simulink model "functional_architecture"  (R2024b)
settings: Solver=VariableStepAuto  StartTime=0.0  StopTime=10.0  RelTol=1e-3
settings Model: Creator=upattacini  LastModifiedBy=mfussi
settings DataIOCC: SaveOutput=off  SignalLogging=off  DSMLogging=off  SaveTime=off
settings RTWCC: GPUComputeCapability=3.5

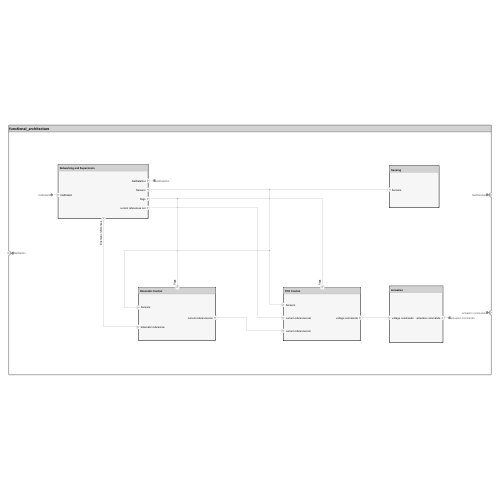
[thumbnail: Simulink's stored preview of the top-level diagram]
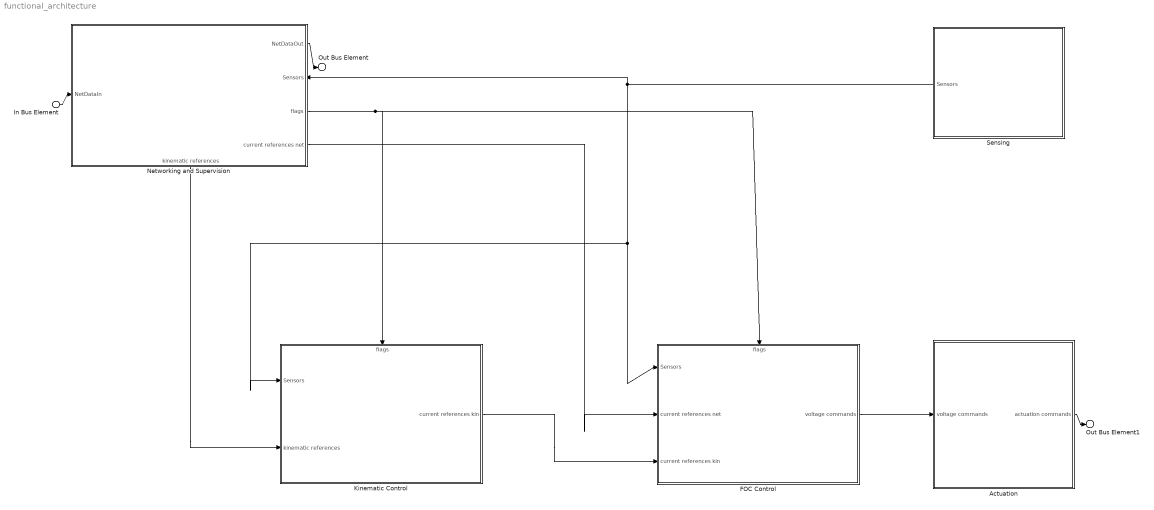
== system functional_architecture ==
  In Bus Element : Inport  PortName=NetDataIn
  Actuation : Subsystem
      settings: PortSchema="{\"entries\":[{\"content\":{\"headerSize\":26,\"margin\":15,\"minimumSpacing\":25,\"sides\":[{\"content\":{\"connectorIds\":[\"In1\"]},\"type\":\"ConnectorPlacement.EquallySpacedRectSide\",\"uuid\":\"e347ee40-d54e-44fd-bc32-f8b024d9ce0e\"},{\"content\":{\"connectorIds\":[\"Out1\"],\"side\":\"RIGHT\"},\"type\":\"ConnectorPlacement.EquallySpacedRectSide\",\"uuid\":\"0804b9f8-7204-402a-a199-b5abf958a170\"},{\"content\":{\"side\":\"TOP\"},\"type\":\"ConnectorPlacement.EquallySpacedRectSide\",\"uuid\":\"09180045-bcf9-4b06-aaa4-a03943964dca\"}]},\"type\":\"ConnectorPlacement.EquallySpacedConnector\",\"uuid\":\"bea07901-0638-4912-923c-a7a96e6d9f8d\"}],\"packageUris\":[\"http://schema.mathworks.com/mf0/Connector/R2020b\"],\"version\":\"1.0\"}"
  FOC Control : Subsystem
      settings: PortSchema="{\"entries\":[{\"content\":{\"headerSize\":26,\"margin\":15,\"minimumSpacing\":25,\"sides\":[{\"content\":{\"connectorIds\":[\"In3\",\"In2\",\"In4\"]},\"type\":\"ConnectorPlacement.EquallySpacedRectSide\",\"uuid\":\"e347ee40-d54e-44fd-bc32-f8b024d9ce0e\"},{\"content\":{\"connectorIds\":[\"Out1\"],\"side\":\"RIGHT\"},\"type\":\"ConnectorPlacement.EquallySpacedRectSide\",\"uuid\":\"0804b9f8-7204-402a-a199-b5abf958a170\"},{\"content\":{\"connectorIds\":[\"In1\"],\"side\":\"TOP\"},\"type\":\"ConnectorPlacement.EquallySpacedRectSide\",\"uuid\":\"09180045-bcf9-4b06-aaa4-a03943964dca\"},{\"content\":{\"side\":\"BOTTOM\"},\"type\":\"ConnectorPlacement.EquallySpacedRectSide\",\"uuid\":\"ba1d2f98-a278-4884-ad0d-7d0295f27101\"}]},\"type\":\"ConnectorPlacement.EquallySpacedConnector\",\"uuid\":\"bea07901-0638-4912-923c-a7a96e6d9f8d\"}],\"packageUris\":[\"http://schema.mathworks.com/mf0/Connector/R2020b\"],\"version\":\"1.0\"}"
  Kinematic Control : Subsystem
      settings: PortSchema="{\"entries\":[{\"content\":{\"headerSize\":26,\"margin\":15,\"minimumSpacing\":25,\"sides\":[{\"content\":{\"connectorIds\":[\"In2\",\"In3\"]},\"type\":\"ConnectorPlacement.EquallySpacedRectSide\",\"uuid\":\"e347ee40-d54e-44fd-bc32-f8b024d9ce0e\"},{\"content\":{\"connectorIds\":[\"Out1\"],\"side\":\"RIGHT\"},\"type\":\"ConnectorPlacement.EquallySpacedRectSide\",\"uuid\":\"0804b9f8-7204-402a-a199-b5abf958a170\"},{\"content\":{\"connectorIds\":[\"In1\"],\"side\":\"TOP\"},\"type\":\"ConnectorPlacement.EquallySpacedRectSide\",\"uuid\":\"09180045-bcf9-4b06-aaa4-a03943964dca\"},{\"content\":{\"side\":\"BOTTOM\"},\"type\":\"ConnectorPlacement.EquallySpacedRectSide\",\"uuid\":\"ba1d2f98-a278-4884-ad0d-7d0295f27101\"}]},\"type\":\"ConnectorPlacement.EquallySpacedConnector\",\"uuid\":\"bea07901-0638-4912-923c-a7a96e6d9f8d\"}],\"packageUris\":[\"http://schema.mathworks.com/mf0/Connector/R2020b\"],\"version\":\"1.0\"}"
  Networking and Supervision : Subsystem
      settings: PortSchema="{\"entries\":[{\"content\":{\"headerSize\":26,\"margin\":15,\"minimumSpacing\":25,\"sides\":[{\"content\":{\"connectorIds\":[\"In2\"]},\"type\":\"ConnectorPlacement.EquallySpacedRectSide\",\"uuid\":\"e347ee40-d54e-44fd-bc32-f8b024d9ce0e\"},{\"content\":{\"connectorIds\":[\"Out4\",\"In1\",\"Out1\",\"Out2\"],\"side\":\"RIGHT\"},\"type\":\"ConnectorPlacement.EquallySpacedRectSide\",\"uuid\":\"0804b9f8-7204-402a-a199-b5abf958a170\"},{\"content\":{\"side\":\"TOP\"},\"type\":\"ConnectorPlacement.EquallySpacedRectSide\",\"uuid\":\"09180045-bcf9-4b06-aaa4-a03943964dca\"},{\"content\":{\"connectorIds\":[\"Out3\"],\"side\":\"BOTTOM\"},\"type\":\"ConnectorPlacement.EquallySpacedRectSide\",\"uuid\":\"f4ab9b4d-91bc-4bf6-80b7-1e0f4f000218\"}]},\"type\":\"ConnectorPlacement.EquallySpacedConnector\",\"uuid\":\"bea07901-0638-4912-923c-a7a96e6d9f8d\"}],\"packageUris\":[\"http://schema.mathworks.com/mf0/Connector/R2020b\"],\"version\":\"1.0\"}"
  Sensing : Subsystem
      settings: PortSchema="{\"entries\":[{\"content\":{\"headerSize\":26,\"margin\":15,\"minimumSpacing\":25,\"sides\":[{\"content\":{\"connectorIds\":[\"Out1\"]},\"type\":\"ConnectorPlacement.EquallySpacedRectSide\",\"uuid\":\"e347ee40-d54e-44fd-bc32-f8b024d9ce0e\"},{\"content\":{\"side\":\"RIGHT\"},\"type\":\"ConnectorPlacement.EquallySpacedRectSide\",\"uuid\":\"0804b9f8-7204-402a-a199-b5abf958a170\"},{\"content\":{\"side\":\"TOP\"},\"type\":\"ConnectorPlacement.EquallySpacedRectSide\",\"uuid\":\"09180045-bcf9-4b06-aaa4-a03943964dca\"}]},\"type\":\"ConnectorPlacement.EquallySpacedConnector\",\"uuid\":\"bea07901-0638-4912-923c-a7a96e6d9f8d\"}],\"packageUris\":[\"http://schema.mathworks.com/mf0/Connector/R2020b\"],\"version\":\"1.0\"}"
  Out Bus Element : Outport  PortName=NetDataOut
  Out Bus Element1 : Outport  Port=2  PortName=actuation commands
  wires:
  In Bus Element/1 -> Networking and Supervision/2(NetDataIn)
  FOC Control/1(voltage commands) -> Actuation/1(voltage commands)
  Sensing/1(Sensors) -> Kinematic Control/2(Sensors), FOC Control/3(Sensors), Networking and Supervision/1(Sensors)
  Networking and Supervision/3(kinematic references) -> Kinematic Control/3(kinematic references)
  Networking and Supervision/1(flags) -> Kinematic Control/1(flags), FOC Control/1(flags)
  Kinematic Control/1(current references kin) -> FOC Control/4(current references kin)
  Networking and Supervision/2(current references net) -> FOC Control/2(current references net)
  Networking and Supervision/4(NetDataOut) -> Out Bus Element/1
  Actuation/1(actuation commands) -> Out Bus Element1/1

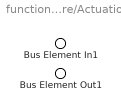
== system functional_architecture/Actuation ==
  Bus Element In1 : Inport  PortName=voltage commands
  Bus Element Out1 : Outport  PortName=actuation commands

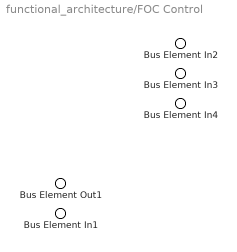
== system functional_architecture/FOC Control ==
  Bus Element In3 : Inport  PortName=flags
  Bus Element In4 : Inport  Port=2  PortName=current references net
  Bus Element In2 : Inport  Port=3  PortName=Sensors
  Bus Element In1 : Inport  Port=4  PortName=current references kin
  Bus Element Out1 : Outport  PortName=voltage commands

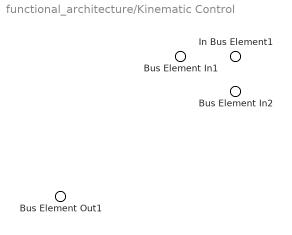
== system functional_architecture/Kinematic Control ==
  Bus Element In1 : Inport  PortName=flags
  In Bus Element1 : Inport  Port=2  PortName=Sensors
  Bus Element In2 : Inport  Port=3  PortName=kinematic references
  Bus Element Out1 : Outport  PortName=current references kin

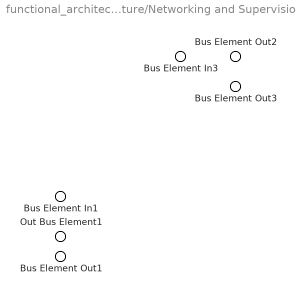
== system functional_architecture/Networking and Supervision ==
  Bus Element In3 : Inport  PortName=Sensors
  Bus Element In1 : Inport  Port=2  PortName=NetDataIn
  Bus Element Out2 : Outport  PortName=flags
  Bus Element Out3 : Outport  Port=2  PortName=current references net
  Bus Element Out1 : Outport  Port=3  PortName=kinematic references
  Out Bus Element1 : Outport  Port=4  PortName=NetDataOut

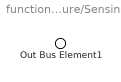
== system functional_architecture/Sensing ==
  Out Bus Element1 : Outport  PortName=Sensors
